simulink model "project"  (R2023b)
settings: Solver=ode45  StartTime=0.0  StopTime=100  RelTol=1e-3  EnableMultiTasking=on
InitFcn:
  | kalmansanszf
values from neighbouring files (symbols this model uses):
  A = [-R/L,       0,    -alpha/L ... (first row only)    [TPintro.m]    (also in kalman.m = zeros(n); kalmansanszf.m = zeros(n))
  C = [0, 1, 0]    [TPintro.m]    (also in kalman.m = [C, zeros(size(C, 1), 1)]; kalmansanszf.m = zeros(2, 11))
  x = zeros(12, 1)    [kalman.m]    (also in kalmansanszf.m = zeros(11, 1))
  x0 = [0.8997 0.8177 0.7215 0.6209 0.5274 0.4498 0.3910 0.3195 0.2418 0.1673 0.1037 0.45]    [CMO_model.m]    (also in CMO_modelp.m = [0.8997 0.8177 0.7215 0.6209 0.5274 0.4498 0.3910 0.3195 0.2; kalman.m = [ 0.8997 0.8177 0.7215 0.6209 0.5274 0.4498 0.3910 0.3195 0.; kalmansanszf.m = [ 0.8997 0.8177 0.7215 0.6209 0.5274 0.4498 0.3910 0.3195 0.)
undefined symbols (not defined in the file or in its folder): Continuous, Time
libraries: simulink x2, ctrlSharedLib x1
settings Model: Creator=busvelle  LastModifiedBy=Lucas
settings SolverCC: AlgebraicLoopSolver=TrustRegion
settings DataIOCC: SaveFormat=Array  SignalLoggingSaveFormat=ModelDataLogs  ReturnWorkspaceOutputs=off
settings OptimizationCC: BlockReduction=off  BooleanDataType=off  ReuseModelBlockBuffer=off  LifeSpan=inf
settings DebuggingCC: SaveWithParameterizedLinksMsg=none  UnderspecifiedInitializationDetection=Classic  MergeDetectMultiDrivingBlocksExec=none  SignalResolutionControl=TryResolveAllWithWarning  MultiTaskDSMMsg=warning  MultiTaskCondExecSysMsg=none  UnconnectedInputMsg=warning  UnconnectedOutputMsg=warning  UnconnectedLineMsg=warning  StateNameClashWarn=warning  SFUnexpectedBacktrackingDiag=warning  SFNoUnconditionalDefaultTransitionDiag=warning  SFExecutionAtInitializationDiag=none  ArithmeticOperatorsInVariantConditions=warning
settings HardwareCC: ProdBitPerPointer=32  ProdBitPerSizeT=32  ProdBitPerPtrDiffT=32  ProdLargestAtomicFloat=None  ProdIntDivRoundTo=Undefined  ProdEndianess=Unspecified  ProdWordSize=32  ProdHWDeviceType=32-bit Generic  TargetUnknown=on
settings ModelReferenceCC: EnableRefExpFcnMdlSchedulingChecks=on  PropagateSignalLabelsOutOfModel=off
settings SFSimCC: SimUseLocalCustomCode=off  CustomCodeUndefinedFunction=UseInterfaceOnly
settings RTWCC: RTWUseLocalCustomCode=off
settings CodeAppCC: StateflowObjectComments=on
settings GRTTargetCC: TargetLangStandard=C89/C90 (ANSI)  CombineOutputUpdateFcns=off  GRTInterface=on
settings ConfigComp: CovMetricSettings=dw  CovSaveCumulativeToWorkspaceVar=on  CovSaveSingleToWorkspaceVar=on  CovExternalEMLEnable=off

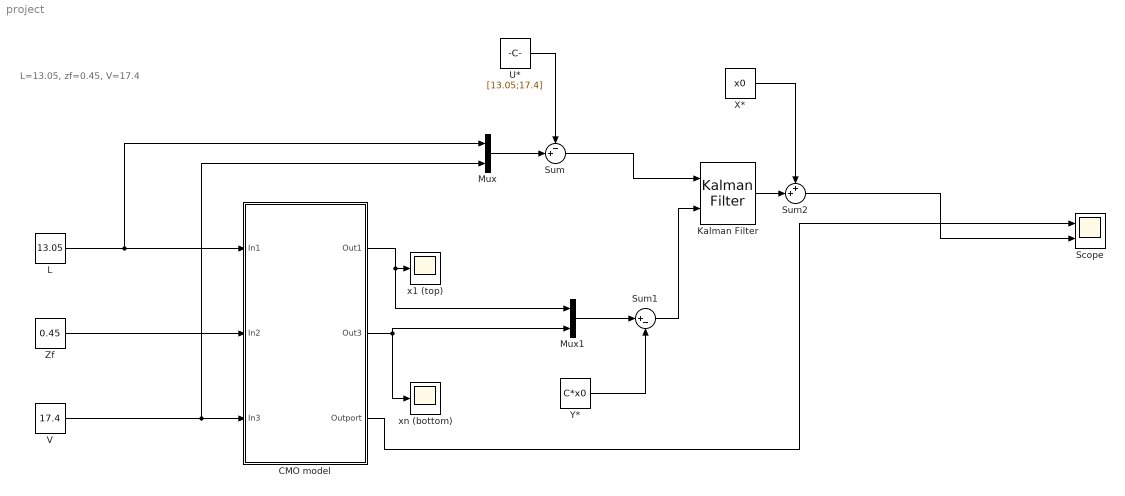
== system project ==
  note: L=13.05, zf=0.45, V=17.4
  CMO model : Subsystem
      mask Display: image('colonne.jpg')
  Kalman Filter : ctrlSharedLib/Kalman Filter  TimeDomain=Continuous-Time  UseCurrentEstimator=on  ModelSource=Individual A, B, C, D matrices  ModelSourceVariable=ss(0.95,1,1,0,1)  A=A  B=B([1:end],[1;end])  C=C  D=0  NumberOfStates=1  NumberOfInputs=1  NumberOfOutputs=1  InitialEstimateSource=Dialog  X0=x  P0=10  UseK=off  UseGH=off  NumberOfProcessNoiseInputs=1  G=1  TimeInvariantG=on  H=0  TimeInvariantH=on  Q=0.1  TimeInvariantQ=on  R=0.00001  TimeInvariantR=on  N=0  TimeInvariantN=on  AddInputPort=on  AddEnablePort=off  OutputEstimatedY=off  OutputP=off  Ts=-1
  L : Constant  Value=13.05
  Mux : Mux  Inputs=2
  Mux1 : Mux  Inputs=2
  Scope : Scope  NumInputPorts=2
  Sum : Sum  Inputs=-+|
  Sum1 : Sum  Inputs=|+-
  Sum2 : Sum  Inputs=++|
  U* : Constant  Value=[13.05;17.4]
  V : Constant  Value=17.4
  X* : Constant  Value=x0
  Y* : Constant  Value=C*x0
  Zf : Constant  Value=0.45
  x1 (top) : Scope
  xn (bottom) : Scope
  wires:
  L/1 -> Mux/1, CMO model/1(In1)
  CMO model/1(Out1) -> Mux1/1, x1 (top)/1
  V/1 -> Mux/2, CMO model/3(In3)
  Zf/1 -> CMO model/2(In2)
  CMO model/2(Out3) -> xn (bottom)/1, Mux1/2
  CMO model/3(Outport) -> Scope/1
  Mux/1 -> Sum/2
  U*/1 -> Sum/1
  Sum/1 -> Kalman Filter/1
  Mux1/1 -> Sum1/1
  Y*/1 -> Sum1/2
  Sum1/1 -> Kalman Filter/2
  Kalman Filter/1 -> Sum2/2
  X*/1 -> Sum2/1
  Sum2/1 -> Scope/2

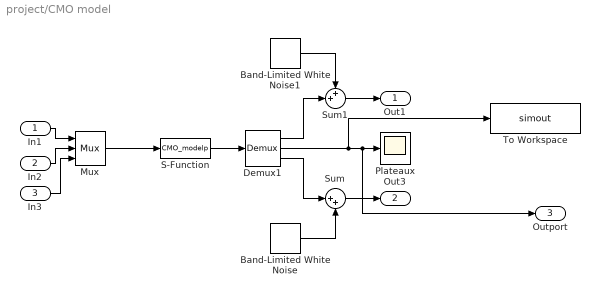
== system project/CMO model ==
  In1 : Inport
  In2 : Inport  Port=2
  In3 : Inport  Port=3
  Band-Limited White Noise : simulink/Sources/Band-Limited White Noise  Cov=[0.0001]  Ts=1  seed=[23341]
  Band-Limited White Noise1 : simulink/Sources/Band-Limited White Noise  Cov=[0.0001]  Ts=1  seed=[23341]
  Demux1 : Demux  Outputs=[1,11,1]
      settings: DisplayOption=none
  Mux : Mux  Inputs=3
  Plateaux : Scope
  S-Function : S-Function  FunctionName=CMO_modelp  SFunctionDeploymentMode=off  EnableBusSupport=off
  Sum : Sum  Inputs=|++
  Sum1 : Sum  Inputs=++|
  To Workspace : ToWorkspace  VariableName=simout  SaveFormat=Timeseries  SampleTime=-1
  Out1 : Outport  InitialOutput=0  VectorParamsAs1DForOutWhenUnconnected=off
  Out3 : Outport  Port=2  VectorParamsAs1DForOutWhenUnconnected=off
  Outport : Outport  Port=3
  wires:
  In3/1 -> Mux/3
  Demux1/2 -> To Workspace/1, Outport/1, Plateaux/1
  S-Function/1 -> Demux1/1
  In2/1 -> Mux/2
  In1/1 -> Mux/1
  Mux/1 -> S-Function/1
  Sum/1 -> Out3/1
  Demux1/3 -> Sum/1
  Band-Limited White Noise/1 -> Sum/2
  Sum1/1 -> Out1/1
  Demux1/1 -> Sum1/2
  Band-Limited White Noise1/1 -> Sum1/1
